simulink model "tec_controller_demo"  (R2025b)
settings: Solver=ode45  StartTime=0.0  StopTime=23400  MaxStep=0.5  RelTol=1e-6
InitFcn:
  | % Define any of these in the base workspace to change them.
  | % Setpoints [t (s), degC]: the standard 15-65 degC calibration sequence, 30 min a step.
  | if ~exist('tec_setpoints', 'var'), tec_setpoints = [(0:12)'*1800, [25 15 25 35 45 55 65 60 50 40 30 20 25]']; end
  | % The crystal reading the loop gets: crystal_scale*(T - 25) + 25 + crystal_offset.
  | % A profile from another crystal reads changes crystal_scale times too large,
  | % which multiplies Kd; the offset does nothing.
  | if ~exist('crystal_scale', 'var'), crystal_scale = 1; end
  | if ~exist('crystal_offset', 'var'), crystal_offset = 0; end
  | % The PT100 reading noise (degC rms, the LTC2986 on rp-f0ea58 shows ~0.013).
  | if ~exist('pt100_noise', 'var'), pt100_noise = 0.013; end
  | % The drive that holds the first setpoint (the holding curve of the TEC holder block),
  | % so the loop starts settled.
  | tec_T0 = tec_setpoints(1, 2);
  | tec_w = (tec_T0 - 22.2)/(1 + 0.0014*(tec_T0 - 22.2));
  | if tec_w >= 0, tec_u0 = (0.495 - sqrt(0.495^2 - 4*0.00067*tec_w))/(2*0.00067);
  | else, tec_u0 = (-0.261 + sqrt(0.261^2 + 4*0.00044*tec_w))/(2*0.00044); end
values from neighbouring files (symbols this model uses):
  PT100 = crystal (64.5 s + 1)/((80.1 s + 1)(6.7 s + 1)).']    [make_tec_holder.m]
undefined symbols (not defined in the file or in its folder): crystal_offset, crystal_scale, pt100_noise
libraries: tec_controller_lib x1, tec_holder_lib x1
Description:
  | The TEC controller block (the Pitaya's TEC loop, tec_controller_block.m) driving the TEC holder block. Choose the source and the gains in the controller's mask; crystal_scale, crystal_offset, pt100_noise and tec_setpoints in the base workspace (see the InitFcn).
settings Model: Creator=wardenaar  LastModifiedBy=wardenaar

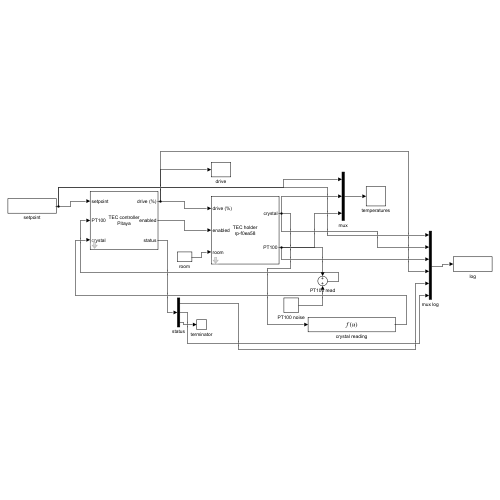
[thumbnail: Simulink's stored preview of the top-level diagram]
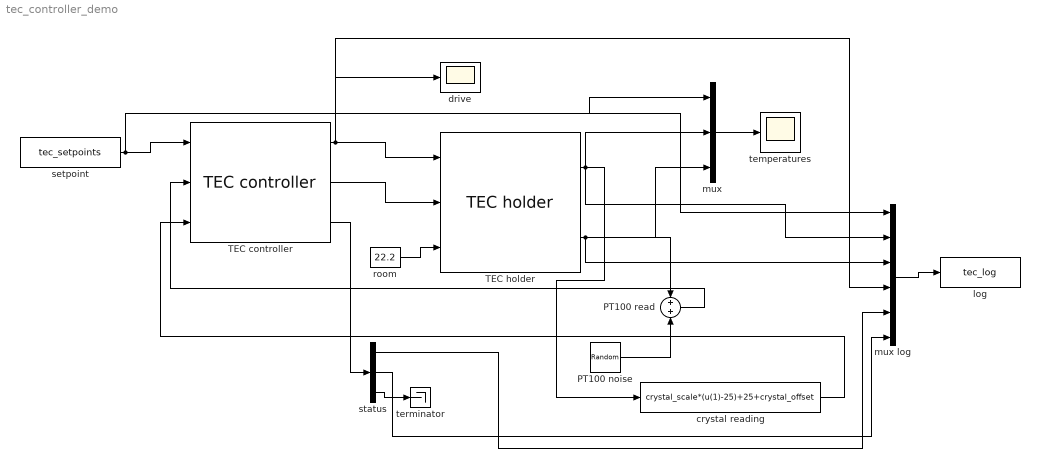
== system tec_controller_demo ==
  PT100 noise : RandomNumber  Variance=pt100_noise^2  Seed=1  SampleTime=1
  PT100 read : Sum
  TEC controller : tec_controller_lib/TEC controller  source=PT100 + crystal for D  kp=39.9  ki=0.196  kd=2000  i_band=1  max_output=100  t_min=5  t_max=75  pt100_s=1  i0=tec_u0
  TEC holder : tec_holder_lib/TEC holder  a=0.495  b=0.00067  c=0.261  d=0.00044  kap=-0.0014  t1=312  t1_off=411  t2=12.2  theta=2.3  z=64.5  ta=80.1  tp=6.7  T0=tec_T0  Ta0=22.2
  crystal reading : Fcn  Expr=crystal_scale*(u(1)-25)+25+crystal_offset
  drive : Scope
  log : ToWorkspace  VariableName=tec_log  SaveFormat=Timeseries  SampleTime=-1
  mux : Mux  Inputs=3
  mux log : Mux  Inputs=6
  room : Constant  Value=22.2
  setpoint : FromWorkspace  VariableName=tec_setpoints  Interpolate=off  OutputAfterFinalValue=Holding final value
  status : Demux  Outputs=3
  temperatures : Scope
  terminator : Terminator
  wires:
  setpoint/1 -> TEC controller/1, mux/1, mux log/1
  PT100 read/1 -> TEC controller/2
  crystal reading/1 -> TEC controller/3
  TEC controller/1 -> TEC holder/1, drive/1, mux log/4
  TEC controller/2 -> TEC holder/2
  room/1 -> TEC holder/3
  TEC holder/2 -> PT100 read/1, mux/3, mux log/3
  PT100 noise/1 -> PT100 read/2
  TEC holder/1 -> crystal reading/1, mux/2, mux log/2
  TEC controller/3 -> status/1
  mux/1 -> temperatures/1
  status/1 -> mux log/5
  status/2 -> mux log/6
  status/3 -> terminator/1
  mux log/1 -> log/1
